simulink model "sens_gnss_model"  (R2026b)
settings: Solver=VariableStepAuto
values from neighbouring files (symbols this model uses):
  D = zeros(nx, ny, 'uint8')    [sens_lidar2d_fast.m]
  P = (P + P.')/2    [sens_nav_ekf.m]
undefined symbols (not defined in the file or in its folder): sens_gnss_fixchain_prm, Ts
libraries: sensorgpslib x3, sharedutil x1
settings Model: Creator=aomar  LastModifiedBy=aomar

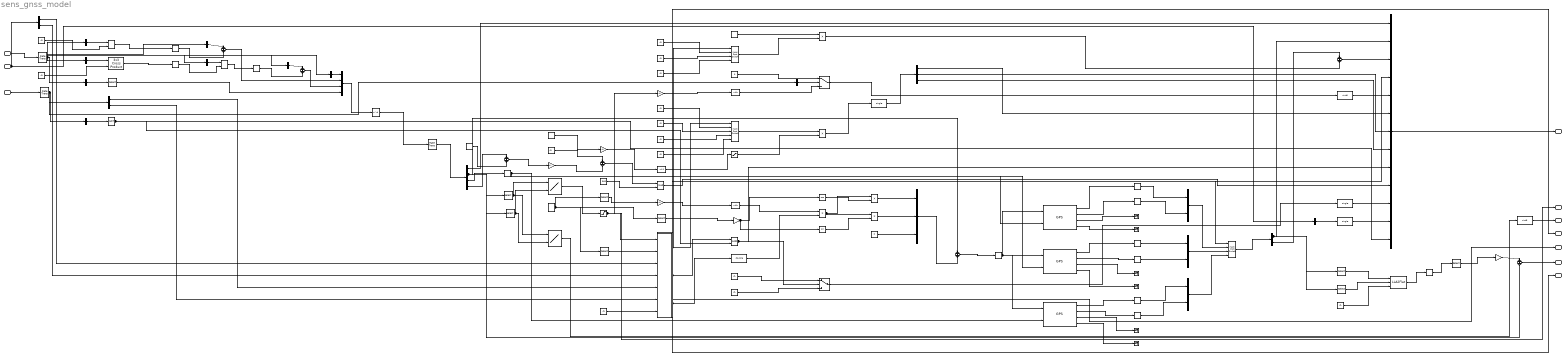
== system sens_gnss_model ==
  truth : Inport  OutDataTypeStr=Bus: Bus_TruthState  SampleTime=Ts.base
  elec_env : Inport  Port=2  OutDataTypeStr=Bus: Bus_ElecEnv  SampleTime=Ts.hk
  flt : Inport  Port=3  OutDataTypeStr=Bus: Bus_FaultInject  SampleTime=Ts.ctrl
  AccOut : Demux  Outputs=3
  AccRep : Product  Inputs=**
  AccSel : MultiPortSwitch  DataPortOrder=Specify indices  Inputs=4  DataPortIndices={4,5,1,0}  DiagnosticForDefault=None  SaturateOnIntegerOverflow=off  InputSameDT=off
  AccSingle : DataTypeConversion  OutDataTypeStr=single  RndMeth=Nearest  SaturateOnIntegerOverflow=off
  Acc_accFixed : Constant  Value=P.sensors.gnss.accFixed  SampleTime=Ts.gnss
  Acc_accFloat : Constant  Value=P.sensors.gnss.accFloat  SampleTime=Ts.gnss
  Acc_accNoFix : Constant  Value=P.sensors.gnss.accNoFix  SampleTime=Ts.gnss
  Acc_accSingle : Constant  Value=P.sensors.gnss.accSingle  SampleTime=Ts.gnss
  Alt : Selector  InputPortWidth=3  IndexOptions=Index vector (dialog)  Indices=3  OutputSizes=1
  AntX : Selector  InputPortWidth=3  IndexOptions=Index vector (dialog)  Indices=1  OutputSizes=1
  AntY : Selector  InputPortWidth=3  IndexOptions=Index vector (dialog)  Indices=2  OutputSizes=1
  BC_Gnss : BusCreator  Inputs=13  OutDataTypeStr=Bus: Bus_GnssRaw  NonVirtualBus=on
      settings: InheritFromInputs=off
  C360 : Constant  Value=360  SampleTime=Ts.gnss
  ChainPrm : Constant  Value=sens_gnss_fixchain_prm(P.sensors.gnss)
  Corr : BusSelector  OutputSignals=gnssCorrOK,gnssCorrAge
  CorrAgeS : DataTypeConversion  OutDataTypeStr=single  RndMeth=Nearest  SaturateOnIntegerOverflow=off
  Corr_gnssCorrAge : BusSelector  OutputSignals=gnssCorrAge
  CosDir : Trigonometry  Operator=cos
  Dir2Pi : Gain  Gain=2*pi
  Epoch : Demux  Outputs=[1 3 3 1]
  FixChain : MATLAB Function  TreatAsAtomicUnit=on
  FixSel : MultiPortSwitch  DataPortOrder=Specify indices  DataPortIndices={4,5,1}  DiagnosticForDefault=None  SaturateOnIntegerOverflow=off  InputSameDT=off
  Flt : BusSelector  OutputSignals=gnss_outage,gnss_force_float
  Flt_gnss_outage : BusSelector  OutputSignals=gnss_outage
  Flt_gnss_outage_2 : BusSelector  OutputSignals=gnss_outage
  GPS_FIXED : sensorgpslib/GPS  DispRefFrame=ENU  PositionInputFormat=Local  ReferenceLocation=P.sensors.refLLA  HorizontalPositionAccuracy=P.sensors.gnss.sigH(1)  VerticalPositionAccuracy=P.sensors.gnss.sigV(1)  VelocityAccuracy=0  DecayFactor=P.sensors.gnss.decay(1)  SeedDouble=P.sensors.gnss.seeds(1)  SimulateUsing=Code generation
      settings: LibrarySourceBlock=mspsensorlib/GPS
  GPS_FLOAT : sensorgpslib/GPS  DispRefFrame=ENU  PositionInputFormat=Local  ReferenceLocation=P.sensors.refLLA  HorizontalPositionAccuracy=P.sensors.gnss.sigH(2)  VerticalPositionAccuracy=P.sensors.gnss.sigV(2)  VelocityAccuracy=0  DecayFactor=P.sensors.gnss.decay(2)  SeedDouble=P.sensors.gnss.seeds(2)  SimulateUsing=Code generation
      settings: LibrarySourceBlock=mspsensorlib/GPS
  GPS_SINGLE : sensorgpslib/GPS  DispRefFrame=ENU  PositionInputFormat=Local  ReferenceLocation=P.sensors.refLLA  HorizontalPositionAccuracy=P.sensors.gnss.sigH(3)  VerticalPositionAccuracy=P.sensors.gnss.sigV(3)  VelocityAccuracy=0  DecayFactor=P.sensors.gnss.decay(3)  SeedDouble=P.sensors.gnss.seeds(3)  SimulateUsing=Code generation
      settings: LibrarySourceBlock=mspsensorlib/GPS
  GpsOut : Demux  Outputs=[3 3]
  Head90 : Constant  Value=90 - P.sensors.gnss.psiBaseline*180/pi  SampleTime=Ts.gnss
  HeadAcc : Switch  Criteria=u2 ~= 0  SaturateOnIntegerOverflow=off  InputSameDT=off
  HeadAccBad : Constant  Value=P.sensors.gnss.headAccInvalid_deg  SampleTime=Ts.gnss
  HeadAccOK : Constant  Value=P.sensors.gnss.head_sigma_deg  SampleTime=Ts.gnss
  HeadAccS : DataTypeConversion  OutDataTypeStr=single  RndMeth=Nearest  SaturateOnIntegerOverflow=off
  HeadCW : Sum  Inputs=+-
  HeadMod : Math  Operator=mod
  HeadNoise : RandomNumber  Variance=P.sensors.gnss.head_sigma^2  Seed=P.sensors.gnss.seedHead  SampleTime=Ts.gnss
  HeadValid : Logic  AllPortsSameDT=off  OutDataTypeStr=boolean
  Href : Constant  Value=-P.sensors.refLLA(3)  SampleTime=Ts.gnss
  Jump : Mux  Inputs=3
  JumpE : Product  Inputs=**
  JumpMag : Product  Inputs=**
  JumpN : Product  Inputs=**
  LLA1d_FIXED : Reshape
  LLA1d_FLOAT : Reshape
  LLA1d_SINGLE : Reshape
  LLA2Flat : LLA2Flat  LL0=P.sensors.refLLA(1:2)
  La_W : Reshape
  LatLon : Selector  InputPortWidth=3  IndexOptions=Index vector (dialog)  Indices=[1 2]  OutputSizes=1
  Latency : Delay  DelayLength=P.sensors.gnss.latencySteps  InitialCondition=0  SampleTime=Ts.ctrl
  MagMin : Bias  Bias=P.sensors.gnss.outlierMag(1)  SaturateOnIntegerOverflow=off
  MagSpan : Gain  Gain=P.sensors.gnss.outlierMag(2) - P.sensors.gnss.outlierMag(1)
  NED1d : Reshape
  NED2ENU : Gain  Gain=[1 1 -1]
  NED2ENU_sel : Selector  InputPortWidth=3  IndexOptions=Index vector (dialog)  Indices=[2 1 3]  OutputSizes=1
  NotOutage : Logic  Operator=NOT  Inputs=1  AllPortsSameDT=off  OutDataTypeStr=boolean
  OmegaXra : sharedutil/3x3 Cross Product  aMode=aMode
      settings: LibrarySourceBlock=aerolibutil/3x3 Cross Product
  Out_FIXED : Mux  Inputs=[3 3]
  Out_FLOAT : Mux  Inputs=[3 3]
  Out_SINGLE : Mux  Inputs=[3 3]
  OutlierD : DataTypeConversion  OutDataTypeStr=double  RndMeth=Nearest  SaturateOnIntegerOverflow=off
  PosAnt : Sum
  PosErr : Sum  Inputs=+-
  PosIn : Sum
  PosRow : Reshape  OutputDimensionality=Row vector (2-D)
  Psi : Selector  InputPortWidth=3  IndexOptions=Index vector (dialog)  Indices=1  OutputSizes=1
  PsiDeg : Gain  Gain=180/pi
  PsiMeas : Sum
  RT_epoch : RateTransition  OutPortSampleTime=Ts.gnss
  RT_flt : RateTransition  OutPortSampleTime=Ts.gnss
  RT_truth : RateTransition  OutPortSampleTime=Ts.ctrl
  RWB_ra : Product  Multiplication=Matrix(*)
  RWB_wxr : Product  Multiplication=Matrix(*)
  RepBias : Bias  Bias=1  SaturateOnIntegerOverflow=off
  RepClamp : Saturate  UpperLimit=P.sensors.gnss.repClamp(2)  LowerLimit=P.sensors.gnss.repClamp(1)
  RepGain : Gain  Gain=P.sensors.gnss.repJitter
  RepNoise : RandomNumber  Seed=P.sensors.gnss.seedJit  SampleTime=Ts.gnss
  SVF_Clamp : Saturate  UpperLimit=P.sensors.gnss.svfClamp(2)  LowerLimit=P.sensors.gnss.svfClamp(1)
  SVF_LUT : Lookup_n-D  BreakpointsForDimension1=P.world.terrain.xE  BreakpointsForDimension2=P.world.terrain.yN  IndexSearchMethod=Evenly spaced points  Table=P.world.gnssSvf  ExtrapMethod=Clip  InternalRulePriority=Speed  RndMeth=Simplest
      settings: InputPortMap=u0,u1
  SV_bias : Bias  Bias=P.sensors.gnss.numSV(1)  SaturateOnIntegerOverflow=off
  SV_gain : Gain  Gain=P.sensors.gnss.numSV(2)
  SV_out : Switch  Criteria=u2 ~= 0  SaturateOnIntegerOverflow=off  InputSameDT=off
  SV_u8 : DataTypeConversion  OutDataTypeStr=uint8  RndMeth=Nearest  SaturateOnIntegerOverflow=off
  SV_zero : Constant  Value=0  SampleTime=Ts.gnss
  SigVel_FIXED : Constant  Value=P.sensors.gnss.sigVel(1)  SampleTime=Ts.gnss
  SigVel_FLOAT : Constant  Value=P.sensors.gnss.sigVel(2)  SampleTime=Ts.gnss
  SigVel_SINGLE : Constant  Value=P.sensors.gnss.sigVel(3)  SampleTime=Ts.gnss
  SinDir : Trigonometry
  TermCrs_FIXED : Terminator
  TermCrs_FLOAT : Terminator
  TermCrs_SINGLE : Terminator
  TermGS_FIXED : Terminator
  TermGS_FLOAT : Terminator
  TermGS_SINGLE : Terminator
  TruthAnt : Mux  Inputs=[1 3 3 1]
  Truth_R_WB : BusSelector  OutputSignals=R_WB
  Truth_R_WB_2 : BusSelector  OutputSignals=R_WB
  Truth_eul : BusSelector  OutputSignals=eul
  Truth_omega_B : BusSelector  OutputSignals=omega_B
  Truth_pos_W : BusSelector  OutputSignals=pos_W
  Truth_t : BusSelector  OutputSignals=t
  Truth_vel_W : BusSelector  OutputSignals=vel_W
  U : UniformRandomNumber  Minimum=zeros(1,6)  Maximum=ones(1,6)  Seed=P.sensors.gnss.seedU  SampleTime=Ts.gnss
  U_chain : Selector  InputPortWidth=6  IndexOptions=Index vector (dialog)  Indices=1:4  OutputSizes=1
  U_dir : Selector  InputPortWidth=6  IndexOptions=Index vector (dialog)  Indices=6  OutputSizes=1
  U_mag : Selector  InputPortWidth=6  IndexOptions=Index vector (dialog)  Indices=5  OutputSizes=1
  Vel1d_FIXED : Reshape
  Vel1d_FLOAT : Reshape
  Vel1d_SINGLE : Reshape
  VelAnt : Sum
  VelMeas : Sum
  VelNoise : RandomNumber  Mean=[0 0 0]  Variance=[1 1 1]  Seed=P.sensors.gnss.seedVel  SampleTime=Ts.gnss
  VelNoiseS : Product  Inputs=**
  VelRow : Reshape  OutputDimensionality=Row vector (2-D)
  VelSigSel : MultiPortSwitch  DataPortOrder=Specify indices  DataPortIndices={4,5,1}  DiagnosticForDefault=None  SaturateOnIntegerOverflow=off  InputSameDT=off
  Wxr_W : Reshape
  Wxr_col : Reshape  OutputDimensionality=Column vector (2-D)
  Zero : Constant  Value=0  SampleTime=Ts.gnss
  ZoneU8 : DataTypeConversion  OutDataTypeStr=uint8  RndMeth=Nearest  SaturateOnIntegerOverflow=off
  Zone_LUT : Lookup_n-D  BreakpointsForDimension1=P.world.terrain.xE  BreakpointsForDimension2=P.world.terrain.yN  IndexSearchMethod=Evenly spaced points  Table=P.world.gnssZoneId  InterpMethod=Nearest  ExtrapMethod=Clip  InternalRulePriority=Speed  RndMeth=Simplest
      settings: InputPortMap=u0,u1
  r_a : Constant  Value=P.sensors.gnss.rAnt1
  r_a_col : Constant  Value=P.sensors.gnss.rAnt1(:)  VectorParams1D=off
  gnss_raw : Outport  OutDataTypeStr=Bus: Bus_GnssRaw
  svf : Outport  Port=2  OutDataTypeStr=double
  zoneId : Outport  Port=3  OutDataTypeStr=uint8
  fixTypeTruth : Outport  Port=4  OutDataTypeStr=uint8
  relposFixed : Outport  Port=5  OutDataTypeStr=boolean
  gnssPosErr : Outport  Port=6  OutDataTypeStr=double
  outlier : Outport  Port=7  OutDataTypeStr=boolean
  wires:
  truth/1 -> RT_truth/1  "truth"
  elec_env/1 -> Corr_gnssCorrAge/1, Corr/1  "elec_env"
  flt/1 -> RT_flt/1  "flt"
  Corr/1 -> FixChain/3(corrOK)  "<gnssCorrOK>"
  Corr/2 -> FixChain/4(corrAge)  "<gnssCorrAge>"
  r_a_col/1 -> RWB_ra/2  "r_a"
  r_a/1 -> OmegaXra/2  "r_a"
  RT_truth/1 -> Truth_eul/1, Truth_t/1, Truth_R_WB/1, Truth_pos_W/1, Truth_vel_W/1, Truth_R_WB_2/1, Truth_omega_B/1  "truth_10ms"
  RT_flt/1 -> Flt_gnss_outage_2/1, Flt/1, Flt_gnss_outage/1  "flt_100ms"
  Truth_R_WB/1 -> RWB_ra/1  "<R_WB>"
  Truth_omega_B/1 -> OmegaXra/1  "<omega_B>"
  Truth_eul/1 -> Psi/1  "<eul>"
  Flt_gnss_outage_2/1 -> NotOutage/1  "<gnss_outage>"
  Flt/1 -> FixChain/5(outage)  "<gnss_outage>"
  Flt/2 -> FixChain/6(forceFloat)  "<gnss_force_float>"
  RWB_ra/1 -> La_W/1  "RWB_ra"
  NotOutage/1 -> HeadValid/2, BC_Gnss/13  "newData"
  Psi/1 -> TruthAnt/4  "psi"
  OmegaXra/1 -> Wxr_col/1  "w_x_ra"
  La_W/1 -> PosAnt/2  "lever_W"
  Wxr_col/1 -> RWB_wxr/2  "Wxr_col"
  Truth_pos_W/1 -> PosAnt/1  "<pos_W>"
  Truth_R_WB_2/1 -> RWB_wxr/1  "<R_WB>"
  PosAnt/1 -> TruthAnt/2  "p_ant"
  RWB_wxr/1 -> Wxr_W/1  "RWB_wxr"
  Wxr_W/1 -> VelAnt/2  "w_x_ra_W"
  Truth_vel_W/1 -> VelAnt/1  "<vel_W>"
  VelAnt/1 -> TruthAnt/3  "v_ant"
  Truth_t/1 -> TruthAnt/1  "<t>"
  TruthAnt/1 -> Latency/1  "ant_truth"
  Latency/1 -> RT_epoch/1  "ant_truth_delayed"
  RT_epoch/1 -> Epoch/1  "ant_epoch"
  Epoch/1 -> BC_Gnss/1  "t_meas"
  Epoch/2 -> PosErr/2, PosIn/1, AntY/1, AntX/1  "p_ant_d"
  Epoch/3 -> VelRow/1  "v_ant_d"
  Epoch/4 -> PsiMeas/1  "psi_d"
  HeadNoise/1 -> PsiMeas/2  "n_head"
  PsiMeas/1 -> PsiDeg/1  "psi_meas"
  VelRow/1 -> GPS_SINGLE/2, GPS_FLOAT/2, GPS_FIXED/2  "VelRow"
  AntX/1 -> Zone_LUT/1, SVF_LUT/1  "x_ant"
  AntY/1 -> Zone_LUT/2, SVF_LUT/2  "y_ant"
  RepNoise/1 -> RepGain/1  "n_rep"
  Head90/1 -> HeadCW/1  "Head90"
  PsiDeg/1 -> HeadCW/2  "psi_deg"
  U/1 -> U_chain/1, U_dir/1, U_mag/1  "u"
  SVF_LUT/1 -> SVF_Clamp/1  "svf_raw"
  Zone_LUT/1 -> ZoneU8/1  "zone_dbl"
  HeadCW/1 -> HeadMod/1  "heading_unwrapped"
  RepGain/1 -> RepBias/1  "RepGain"
  C360/1 -> HeadMod/2  "C360"
  SVF_Clamp/1 -> SV_gain/1, FixChain/1(svf), svf/1  "svf"
  ChainPrm/1 -> FixChain/7(c)  "chain_prm"
  U_mag/1 -> MagSpan/1  "u_mag"
  U_chain/1 -> FixChain/2(u)  "u_chain"
  SigVel_FIXED/1 -> VelSigSel/2  "sigVel_FIXED"
  SigVel_FLOAT/1 -> VelSigSel/3  "sigVel_FLOAT"
  SigVel_SINGLE/1 -> VelSigSel/4  "sigVel_SINGLE"
  SV_gain/1 -> SV_bias/1  "SV_gain"
  Acc_accFixed/1 -> AccSel/2  "Acc_accFixed"
  Acc_accFloat/1 -> AccSel/3  "Acc_accFloat"
  Acc_accSingle/1 -> AccSel/4  "Acc_accSingle"
  Acc_accNoFix/1 -> AccSel/5  "Acc_accNoFix"
  HeadMod/1 -> BC_Gnss/10  "heading_deg"
  MagSpan/1 -> MagMin/1  "MagSpan"
  RepBias/1 -> RepClamp/1  "RepBias"
  U_dir/1 -> Dir2Pi/1  "u_dir"
  VelNoise/1 -> VelNoiseS/1  "n_vel"
  SV_zero/1 -> SV_out/1  "SV_zero"
  RepClamp/1 -> AccRep/2  "k_rep"
  HeadValid/1 -> BC_Gnss/9, HeadAcc/2  "headingValid"
  HeadAccOK/1 -> HeadAcc/1  "HeadAccOK"
  HeadAccBad/1 -> HeadAcc/3  "HeadAccBad"
  VelSigSel/1 -> VelNoiseS/2  "sig_vel"
  AccSel/1 -> AccRep/1  "acc_fix"
  SV_bias/1 -> SV_out/3  "numSV_dbl"
  MagMin/1 -> JumpMag/1  "jump"
  Dir2Pi/1 -> CosDir/1, SinDir/1  "dir"
  OutlierD/1 -> JumpMag/2  "outlier_d"
  Flt_gnss_outage/1 -> SV_out/2  "<gnss_outage>"
  VelNoiseS/1 -> VelMeas/2  "vel_noise"
  AccRep/1 -> AccSingle/1  "acc_rep"
  CosDir/1 -> JumpE/2  "CosDir"
  JumpMag/1 -> JumpE/1, JumpN/1  "jump_on"
  SinDir/1 -> JumpN/2  "SinDir"
  SV_out/1 -> SV_u8/1  "SV_out"
  HeadAcc/1 -> HeadAccS/1  "HeadAcc"
  JumpE/1 -> Jump/1  "JumpE"
  JumpN/1 -> Jump/2  "JumpN"
  Zero/1 -> Jump/3  "Zero"
  AccSingle/1 -> AccOut/1  "AccSingle"
  AccOut/1 -> BC_Gnss/6  "hAcc"
  AccOut/2 -> BC_Gnss/7  "vAcc"
  AccOut/3 -> BC_Gnss/8  "sAcc"
  Jump/1 -> PosIn/2  "jump_ENU"
  PosIn/1 -> PosRow/1  "p_in"
  PosRow/1 -> GPS_SINGLE/1, GPS_FIXED/1, GPS_FLOAT/1  "PosRow"
  GPS_FIXED/1 -> LLA1d_FIXED/1  "lla_FIXED"
  GPS_FIXED/2 -> Vel1d_FIXED/1  "vel_FIXED"
  GPS_FIXED/3 -> TermGS_FIXED/1  "groundspeed_FIXED"
  GPS_FIXED/4 -> TermCrs_FIXED/1  "course_FIXED"
  GPS_FLOAT/1 -> LLA1d_FLOAT/1  "lla_FLOAT"
  GPS_FLOAT/2 -> Vel1d_FLOAT/1  "vel_FLOAT"
  GPS_FLOAT/3 -> TermGS_FLOAT/1  "groundspeed_FLOAT"
  GPS_FLOAT/4 -> TermCrs_FLOAT/1  "course_FLOAT"
  GPS_SINGLE/1 -> LLA1d_SINGLE/1  "lla_SINGLE"
  GPS_SINGLE/2 -> Vel1d_SINGLE/1  "vel_SINGLE"
  GPS_SINGLE/3 -> TermGS_SINGLE/1  "groundspeed_SINGLE"
  GPS_SINGLE/4 -> TermCrs_SINGLE/1  "course_SINGLE"
  LLA1d_FIXED/1 -> Out_FIXED/1  "LLA1d_FIXED"
  Vel1d_FIXED/1 -> Out_FIXED/2  "Vel1d_FIXED"
  LLA1d_FLOAT/1 -> Out_FLOAT/1  "LLA1d_FLOAT"
  Vel1d_FLOAT/1 -> Out_FLOAT/2  "Vel1d_FLOAT"
  LLA1d_SINGLE/1 -> Out_SINGLE/1  "LLA1d_SINGLE"
  Vel1d_SINGLE/1 -> Out_SINGLE/2  "Vel1d_SINGLE"
  Out_FIXED/1 -> FixSel/2  "gps_FIXED"
  Out_FLOAT/1 -> FixSel/3  "gps_FLOAT"
  Out_SINGLE/1 -> FixSel/4  "gps_SINGLE"
  FixSel/1 -> GpsOut/1  "gps_sel"
  GpsOut/1 -> BC_Gnss/2, Alt/1, LatLon/1  "lla"
  GpsOut/2 -> VelMeas/1  "vel_gps"
  Corr_gnssCorrAge/1 -> CorrAgeS/1  "<gnssCorrAge>"
  VelMeas/1 -> BC_Gnss/3  "vel_ENU"
  Href/1 -> LLA2Flat/3  "href"
  LatLon/1 -> LLA2Flat/1  "latlon"
  Alt/1 -> LLA2Flat/2  "h"
  SV_u8/1 -> BC_Gnss/5  "numSV"
  HeadAccS/1 -> BC_Gnss/11  "headAcc_deg"
  CorrAgeS/1 -> BC_Gnss/12  "corrAge"
  BC_Gnss/1 -> gnss_raw/1  "gnss_raw"
  LLA2Flat/1 -> NED1d/1  "p_NED"
  NED1d/1 -> NED2ENU_sel/1  "NED1d"
  NED2ENU_sel/1 -> NED2ENU/1  "NED2ENU_sel"
  NED2ENU/1 -> PosErr/1  "p_rep_ENU"
  PosErr/1 -> gnssPosErr/1  "gnssPosErr"
  ZoneU8/1 -> zoneId/1  "zoneId"
  FixChain/1(fixType) -> VelSigSel/1, BC_Gnss/4, AccSel/1, fixTypeTruth/1, FixSel/1  "fixType"
  FixChain/2(relposFixed) -> HeadValid/1, relposFixed/1  "relposFixed"
  FixChain/3(outlier) -> OutlierD/1, outlier/1  "outlier"

== matlab function sens_gnss_model/FixChain ==
  settings: description=RTK fix-state Markov chain (sensors spec 3.2, F2): subsystems/sensors/sens_gnss_fixchain.m; input c = sens_gnss_fixchain_prm(P.sensors.gnss)
  data: svf input; u input; fixType output; corrOK input; corrAge input; outage input; forceFloat input; c input; relposFixed output; outlier output
function [fixType, relposFixed, outlier] = fcn(svf, u, corrOK, corrAge, outage, forceFloat, c)
%#codegen
[fixType, relposFixed, outlier] = sens_gnss_fixchain(svf, u, corrOK, corrAge, outage, forceFloat, c);
